simulink model "KUKA_main_simmechanic"  (R2015a)
settings: Solver=ode45  StartTime=0.0  StopTime=61.2  RelTol=1e-3
undefined symbols (not defined in the file or in its folder): KUKA, part1, part2, part3, part4, RootGround, RootPart, sfun3d
libraries: mblibv1 x16
settings Model: Creator=PHANTU  LastModifiedBy=PHANTU
settings SimMechanicsCC: VisOnUpdateDiagram=on  VisDuringSimulation=on

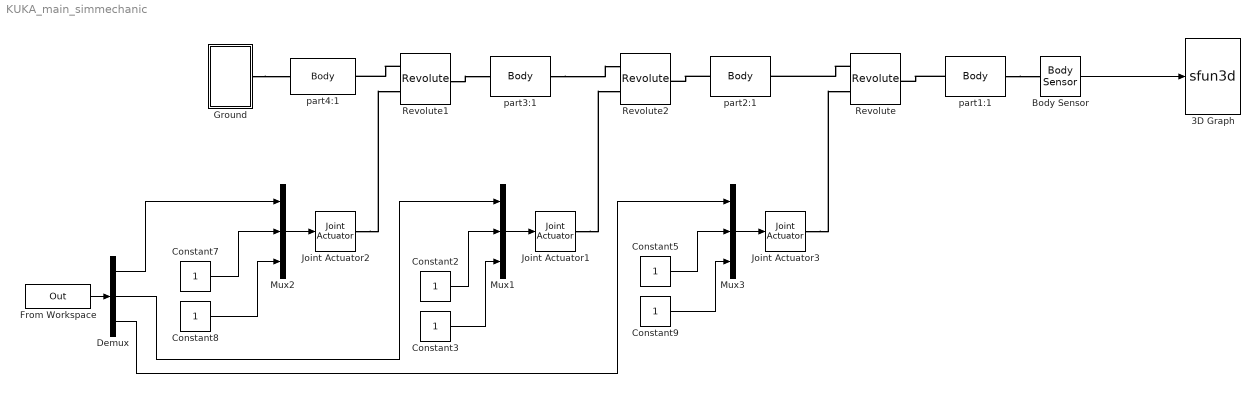
== system KUKA_main_simmechanic ==
  3D Graph : S-Function  LoadFcn=sfun3d([],[],[],'LoadBlock')  StartFcn=sfun3d([],[],[],'Start')  StopFcn=sfun3d([],[],[],'Stop')  FunctionName=sfun3d  Parameters=ax,T,np,cp,gd,ls,mk  mask(3D Graph){np=1, ax=[-50 800 -50 800 -100 800], cp=[40000 0 -50], gd=on, ls=-, mk=none, T=-1}
      mask prompts: np "Number of point (lines)"; ax "[xmin xmax  ymin ymax zmin zmax]"; cp "Camera position (use [0 0 1] for 2D XY view)"; gd "Grid (on|off)"; ls "LineStyle"; mk "Marker"; T "Sampling Time"
      mask help:
      | This block plots the position of several points in the XYZ space. The input contains the coordinates of all the points (x1,y1,z1,x2,y2,z2,...).
      | The number of points (lines), the XYZ ranges, camera position, grid, linestyle, marker and sampling time, can be set as mask parameters.
      settings: CopyFcn=sfun3d([],[],[],'CopyBlock')  DeleteFcn=sfun3d([],[],[],'DeleteBlock')  NameChangeFcn=sfun3d([],[],[],'NameChange')
      mask Help:
      | This block plots the position of several points in the XYZ space. The input contains the coordinates of all the points (x1,y1,z1,x2,y2,z2,...).
      | The number of points (lines), the XYZ ranges, camera position, grid, linestyle, marker and sampling time, can be set as mask parameters.
      mask TypeOptions ls: - | -- | : | -. | none
      mask TypeOptions mk: none | . | + | o | * | x | square | diamond | v | ^ | > | < | pentagram | hexagram
      mask Display: plot([.05 .95 .95 .05 .05],[.45 .45 .95 .95 .45], 0.5+cos(0:0.1:2*pi)*0.3,0.7+sin(0:0.1:2*pi)*0.2)
  Body Sensor : mblibv1/Sensors &  Actuators/Body Sensor  UpdateFromCAD=off  PhysicalDomain=Mechanical  PortType=blob  Muxed=on  Pose=off  Angle=on  AngleUnits=deg  ArcVelocity=off  ArcVelocityUnits=deg/s  ArcAcceleration=off  ArcAccelerationUnits=deg/s^2  CoordPosition=on  CoordPositionUnits=mm  Velocity=off  VelocityUnits=m/s  Acceleration=off  AccelerationUnits=m/s^2  Quaternion=on  QuaternionDT=off  QuaternionDDT=off  QuaternionUnits=off  OutputVector=[1]  ActiveIO=on  Width=3  DialogClass=MechanicalSensorBlock  ReferenceFrame=Absolute (World)
  Constant{2..3,5,7..9} (6 alike) : Constant
  Demux : Demux  Outputs=3
  From Workspace : FromWorkspace  VariableName=Out  SampleTime=0.1
  Ground : Subsystem
  Joint Actuator1 : mblibv1/Sensors &  Actuators/Joint Actuator  UpdateFromCAD=off  PhysicalDomain=Mechanical  PortType=blob  ActuationStyle=Motion  AngleUnits=deg  ArcVelocityUnits=deg/s  ArcAccelerationUnits=deg/s^2  CoordPositionUnits=m  VelocityUnits=m/s  AccelerationUnits=m/s^2  ForceUnits=N  TorqueUnits=N*m  ActiveIO=on  Width=3  DialogClass=MechanicalActuatorBlock  Primitive=R1  ReferenceFrame=Absolute (World)
  Joint Actuator2 : mblibv1/Sensors &  Actuators/Joint Actuator  UpdateFromCAD=off  PhysicalDomain=Mechanical  PortType=blob  ActuationStyle=Motion  AngleUnits=deg  ArcVelocityUnits=deg/s  ArcAccelerationUnits=deg/s^2  CoordPositionUnits=m  VelocityUnits=m/s  AccelerationUnits=m/s^2  ForceUnits=N  TorqueUnits=N*m  ActiveIO=on  Width=3  DialogClass=MechanicalActuatorBlock  Primitive=R1  ReferenceFrame=Absolute (World)
  Joint Actuator3 : mblibv1/Sensors &  Actuators/Joint Actuator  UpdateFromCAD=off  PhysicalDomain=Mechanical  PortType=blob  ActuationStyle=Motion  AngleUnits=deg  ArcVelocityUnits=deg/s  ArcAccelerationUnits=deg/s^2  CoordPositionUnits=m  VelocityUnits=m/s  AccelerationUnits=m/s^2  ForceUnits=N  TorqueUnits=N*m  ActiveIO=on  Width=3  DialogClass=MechanicalActuatorBlock  Primitive=R1  ReferenceFrame=Absolute (World)
  Mux1 : Mux  Inputs=3
  Mux2 : Mux  Inputs=3
  Mux3 : Mux  Inputs=3
  Revolute : mblibv1/Joints/Revolute  LConnTagsString=__newl0|SA1  RConnTagsString=__newr0  UpdateFromCAD=on  PMImportedID=part1:1:-:part2:1  NumSAPorts=1  CutJoint=off  MarkAsCut=off  Primitives=prismatic  PrimitiveProps=R1$World$[0,1,0]$revolute  DialogClass=JointBlock  R1Axis=[0,1,0]
  Revolute1 : mblibv1/Joints/Revolute  LConnTagsString=__newl0|SA1  RConnTagsString=__newr0  UpdateFromCAD=on  PMImportedID=part3:1:-:part4:1  NumSAPorts=1  CutJoint=off  MarkAsCut=off  Primitives=prismatic  PrimitiveProps=R1$World$[0,0,1]$revolute  DialogClass=JointBlock  R1Axis=[0,0,1]
  Revolute2 : mblibv1/Joints/Revolute  LConnTagsString=__newl0|SA1  RConnTagsString=__newr0  UpdateFromCAD=on  PMImportedID=part2:1:-:part3:1  NumSAPorts=1  CutJoint=off  MarkAsCut=off  Primitives=prismatic  PrimitiveProps=R1$World$[0,1,0]$revolute  DialogClass=JointBlock  R1Axis=[0,1,0]
  part1:1 : mblibv1/Bodies/Body  LConnTagsString=CS2  RConnTagsString=CS3  UpdateFromCAD=on  PMImportedID=part1:1  DialogClass=MechanicalBodyBlock  Mass=40.4989  MassUnits=kg  InertiaUnits=kg*m^2  Inertia=[0.772378,0.243082,0.407747;0.243082,3.65301,-0.170622;0.407747,-0.170622,3.50439]  Shape=Cylinder  ShapeDims=[1 1]  ShapeUnits=m  ShapeUse=false  Density=1  DensityUnits=kg/m^3  DensityUse=false  GraphicsMode=GFXFILE  GraphicsFileName=part1_ipt_86567821.STL  BodyColorSelMode=COLORPALETTE  BodyColor=[1;1;0]  AttachedToCS=CS1  CG=Right$CG$[1017.65 45.7629 740.059]$WORLD$WORLD$mm$[1 0 0;0 1 0;0 0 1]$3x3 Transform$rad$WORLD$false$part1:1::CG(AUTOGEN)  WorkingFrames=Right$CS1$[680 0 -679.99]$WORLD$WORLD$mm$[1 0 0;0 1 0;0 0 1]$3x3 Transform$rad$WORLD$false$part1:1::CS1(AUTOGEN)#Left$CS2$[940 -107 675.01]$WORLD$WORLD$mm$[1 0 0;0 1 0;0 0 1]$3x3 Transform$rad$WORLD$true$part1:1:-:part2:1::part1:1(AUTOGEN)#Right$CS3$[1768 0 675.01]$WORLD$WORLD$mm$[1 0 0;0 1 0;0 0 1]$3x3 Transform$rad$WORLD$true$none  CGPos=[1017.65 45.7629 740.059]  CGRot=[1 0 0;0 1 0;0 0 1]  CS0Pos=[]  CS0Rot=[]  CS1Pos=[680 0 -679.99]  CS1Rot=[1 0 0;0 1 0;0 0 1]  CS2Pos=[940 -107 675.01]  CS2Rot=[1 0 0;0 1 0;0 0 1]  CS3Pos=[1768 0 675.01]  CS3Rot=[1 0 0;0 1 0;0 0 1]  CS4Pos=[]  CS4Rot=[]  CS5Pos=[]  CS5Rot=[]  CS6Pos=[]  CS6Rot=[]  CS7Pos=[]  CS7Rot=[]  CS8Pos=[]  CS8Rot=[]  CS9Pos=[]  CS9Rot=[]  CS10Pos=[]  CS10Rot=[]  CS11Pos=[]  CS11Rot=[]  CS12Pos=[]  CS12Rot=[]  CS13Pos=[]  CS13Rot=[]  CS14Pos=[]  CS14Rot=[]  CS15Pos=[]  CS15Rot=[]  CS16Pos=[]  CS16Rot=[]  CS17Pos=[]  CS17Rot=[]  CS18Pos=[]  CS18Rot=[]  CS19Pos=[]  CS19Rot=[]  CS20Pos=[]  CS20Rot=[]
  part2:1 : mblibv1/Bodies/Body  LConnTagsString=CS3  RConnTagsString=CS2  UpdateFromCAD=on  PMImportedID=part2:1  DialogClass=MechanicalBodyBlock  Mass=13.5189  MassUnits=kg  InertiaUnits=kg*m^2  Inertia=[0.595755,-0.000241052,-0.000341583;-0.000241052,0.593927,0.0264066;-0.000341583,0.0264066,0.0592214]  Shape=Cylinder  ShapeDims=[1 1]  ShapeUnits=m  ShapeUse=false  Density=1  DensityUnits=kg/m^3  DensityUse=false  GraphicsMode=GFXFILE  GraphicsFileName=part2_ipt_86567821.STL  BodyColorSelMode=COLORPALETTE  BodyColor=[0;0;1]  AttachedToCS=CS1  CG=Right$CG$[581.389 -180.551 674.773]$WORLD$WORLD$mm$[0 0 1;0 1 0;-1 0 0]$3x3 Transform$rad$WORLD$false$part2:1::CG(AUTOGEN)  WorkingFrames=Right$CS1$[-415 0 935.01]$WORLD$WORLD$mm$[0 0 1;0 1 0;-1 0 0]$3x3 Transform$rad$WORLD$false$part2:1::CS1(AUTOGEN)#Right$CS2$[940 -107 675.01]$WORLD$WORLD$mm$[1 0 0;0 1 0;0 0 1]$3x3 Transform$rad$WORLD$true$part1:1:-:part2:1::part2:1(AUTOGEN)#Left$CS3$[260 -83 675.01]$WORLD$WORLD$mm$[1 0 0;0 1 0;0 0 1]$3x3 Transform$rad$WORLD$true$part2:1:-:part3:1::part2:1(AUTOGEN)  CGPos=[581.389 -180.551 674.773]  CGRot=[0 0 1;0 1 0;-1 0 0]  CS0Pos=[]  CS0Rot=[]  CS1Pos=[-415 0 935.01]  CS1Rot=[0 0 1;0 1 0;-1 0 0]  CS2Pos=[940 -107 675.01]  CS2Rot=[1 0 0;0 1 0;0 0 1]  CS3Pos=[260 -83 675.01]  CS3Rot=[1 0 0;0 1 0;0 0 1]  CS4Pos=[]  CS4Rot=[]  CS5Pos=[]  CS5Rot=[]  CS6Pos=[]  CS6Rot=[]  CS7Pos=[]  CS7Rot=[]  CS8Pos=[]  CS8Rot=[]  CS9Pos=[]  CS9Rot=[]  CS10Pos=[]  CS10Rot=[]  CS11Pos=[]  CS11Rot=[]  CS12Pos=[]  CS12Rot=[]  CS13Pos=[]  CS13Rot=[]  CS14Pos=[]  CS14Rot=[]  CS15Pos=[]  CS15Rot=[]  CS16Pos=[]  CS16Rot=[]  CS17Pos=[]  CS17Rot=[]  CS18Pos=[]  CS18Rot=[]  CS19Pos=[]  CS19Rot=[]  CS20Pos=[]  CS20Rot=[]
  part3:1 : mblibv1/Bodies/Body  LConnTagsString=CS2  RConnTagsString=CS3  UpdateFromCAD=on  PMImportedID=part3:1  DialogClass=MechanicalBodyBlock  Mass=28.3532  MassUnits=kg  InertiaUnits=kg*m^2  Inertia=[1.07185,-0.0539717,-0.354129;-0.0539717,1.05703,-0.0608066;-0.354129,-0.0608066,1.30191]  Shape=Cylinder  ShapeDims=[1 1]  ShapeUnits=m  ShapeUse=false  Density=1  DensityUnits=kg/m^3  DensityUse=false  GraphicsMode=GFXFILE  GraphicsFileName=part3_ipt_86567821.STL  BodyColorSelMode=COLORPALETTE  BodyColor=[1;0.843137;0]  AttachedToCS=CS1  CG=Right$CG$[107.444 17.0185 548.784]$WORLD$WORLD$mm$[1 0 0;0 1 0;0 0 1]$3x3 Transform$rad$WORLD$false$part3:1::CG(AUTOGEN)  WorkingFrames=Right$CS1$[0 0 0.00950136]$WORLD$WORLD$mm$[1 0 0;0 1 0;0 0 1]$3x3 Transform$rad$WORLD$false$part3:1::CS1(AUTOGEN)#Left$CS2$[0 0 396.933]$WORLD$WORLD$mm$[1 0 0;0 1 0;0 0 1]$3x3 Transform$rad$WORLD$true$part3:1:-:part4:1::part3:1(AUTOGEN)#Right$CS3$[260 -83 675.01]$WORLD$WORLD$mm$[1 0 0;0 1 0;0 0 1]$3x3 Transform$rad$WORLD$true$part2:1:-:part3:1::part3:1(AUTOGEN)  CGPos=[107.444 17.0185 548.784]  CGRot=[1 0 0;0 1 0;0 0 1]  CS0Pos=[]  CS0Rot=[]  CS1Pos=[0 0 0.00950136]  CS1Rot=[1 0 0;0 1 0;0 0 1]  CS2Pos=[0 0 396.933]  CS2Rot=[1 0 0;0 1 0;0 0 1]  CS3Pos=[260 -83 675.01]  CS3Rot=[1 0 0;0 1 0;0 0 1]  CS4Pos=[]  CS4Rot=[]  CS5Pos=[]  CS5Rot=[]  CS6Pos=[]  CS6Rot=[]  CS7Pos=[]  CS7Rot=[]  CS8Pos=[]  CS8Rot=[]  CS9Pos=[]  CS9Rot=[]  CS10Pos=[]  CS10Rot=[]  CS11Pos=[]  CS11Rot=[]  CS12Pos=[]  CS12Rot=[]  CS13Pos=[]  CS13Rot=[]  CS14Pos=[]  CS14Rot=[]  CS15Pos=[]  CS15Rot=[]  CS16Pos=[]  CS16Rot=[]  CS17Pos=[]  CS17Rot=[]  CS18Pos=[]  CS18Rot=[]  CS19Pos=[]  CS19Rot=[]  CS20Pos=[]  CS20Rot=[]
  part4:1 : mblibv1/Bodies/Body  LConnTagsString=CS2  RConnTagsString=CS3  UpdateFromCAD=on  PMImportedID=part4:1  DialogClass=MechanicalBodyBlock  Mass=69.1518  MassUnits=kg  InertiaUnits=kg*m^2  Inertia=[1.73395,-0.0485512,-0.0688783;-0.0485512,2.09396,-0.000359291;-0.0688783,-0.000359291,2.19578]  Shape=Cylinder  ShapeDims=[1 1]  ShapeUnits=m  ShapeUse=false  Density=1  DensityUnits=kg/m^3  DensityUse=false  GraphicsMode=GFXFILE  GraphicsFileName=part4_ipt_86567821.STL  BodyColorSelMode=COLORPALETTE  BodyColor=[1;0;0]  AttachedToCS=CS1  CG=Right$CG$[-41.1494 -3.79313 198.366]$WORLD$WORLD$mm$[1 0 0;0 1 0;0 0 1]$3x3 Transform$rad$WORLD$false$part4:1::CG(AUTOGEN)  WorkingFrames=Right$CS1$[0.557964 0.1152 -1.667]$WORLD$WORLD$mm$[1 0 0;0 1 0;0 0 1]$3x3 Transform$rad$WORLD$false$part4:1::CS1(AUTOGEN)#Left$CS2$[0 0 0]$WORLD$WORLD$mm$[1 0 0;0 1 0;0 0 1]$3x3 Transform$rad$WORLD$true$:-:KUKA/RootPart::part4:1(AUTOGEN)#Right$CS3$[0 0 396.933]$WORLD$WORLD$mm$[1 0 0;0 1 0;0 0 1]$3x3 Transform$rad$WORLD$true$part3:1:-:part4:1::part4:1(AUTOGEN)  CGPos=[-41.1494 -3.79313 198.366]  CGRot=[1 0 0;0 1 0;0 0 1]  CS0Pos=[]  CS0Rot=[]  CS1Pos=[0.557964 0.1152 -1.667]  CS1Rot=[1 0 0;0 1 0;0 0 1]  CS2Pos=[0 0 0]  CS2Rot=[1 0 0;0 1 0;0 0 1]  CS3Pos=[0 0 396.933]  CS3Rot=[1 0 0;0 1 0;0 0 1]  CS4Pos=[]  CS4Rot=[]  CS5Pos=[]  CS5Rot=[]  CS6Pos=[]  CS6Rot=[]  CS7Pos=[]  CS7Rot=[]  CS8Pos=[]  CS8Rot=[]  CS9Pos=[]  CS9Rot=[]  CS10Pos=[]  CS10Rot=[]  CS11Pos=[]  CS11Rot=[]  CS12Pos=[]  CS12Rot=[]  CS13Pos=[]  CS13Rot=[]  CS14Pos=[]  CS14Rot=[]  CS15Pos=[]  CS15Rot=[]  CS16Pos=[]  CS16Rot=[]  CS17Pos=[]  CS17Rot=[]  CS18Pos=[]  CS18Rot=[]  CS19Pos=[]  CS19Rot=[]  CS20Pos=[]  CS20Rot=[]
  wires:
  Mux2/1 -> Joint Actuator2/1
  Constant7/1 -> Mux2/2
  Constant8/1 -> Mux2/3
  Mux1/1 -> Joint Actuator1/1
  Constant2/1 -> Mux1/2
  Constant3/1 -> Mux1/3
  Mux3/1 -> Joint Actuator3/1
  Constant5/1 -> Mux3/2
  Constant9/1 -> Mux3/3
  From Workspace/1 -> Demux/1
  Demux/1 -> Mux2/1
  Demux/2 -> Mux1/1
  Demux/3 -> Mux3/1
  Body Sensor/1 -> 3D Graph/1
  connections:
  Revolute1/LConn1 -- part4:1/RConn1
  Revolute1/RConn1 -- part3:1/LConn1
  part3:1/RConn1 -- Revolute2/LConn1
  Revolute/LConn1 -- part2:1/RConn1
  part2:1/LConn1 -- Revolute2/RConn1
  part1:1/LConn1 -- Revolute/RConn1
  Ground/RConn1 -- part4:1/LConn1
  Joint Actuator2/RConn1 -- Revolute1/LConn2
  Joint Actuator1/RConn1 -- Revolute2/LConn2
  Joint Actuator3/RConn1 -- Revolute/LConn2
  part1:1/RConn1 -- Body Sensor/LConn1

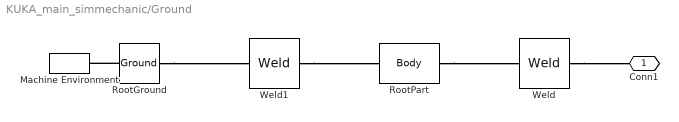
== system KUKA_main_simmechanic/Ground ==
  Machine Environment : mblibv1/Bodies/Machine Environment  PortType=env  PhysicalDomain=Mechanical  DialogTemplateClass=MECH.MachineEnvironment  SyncWhenCopied=off  Gravity=[0 0 -9.81]  GravityUnits=m/s^2  GravityAsSignal=off  Dimensionality=Auto-detect  AnalysisType=Forward dynamics  LinearAssemblyTolerance=1e-3  LinearAssemblyToleranceUnits=m  AngularAssemblyTolerance=1e-3  AngularAssemblyToleranceUnits=rad  ConstraintSolverType=Stabilizing  ConstraintRelTolerance=1e-4  ConstraintAbsTolerance=1e-4  UseRobustSingularityHandling=off  RedundancyAnalysisToleranceType=Automatically select tolerance  RedundancyAnalysisTolerance=1e-14  StatePerturbationType=Fixed  PerturbationSize=1e-5  VisualizeMachine=on  BodyVisualizationType=Use model default body geometries  BodyColorSelMode=Use model default  DefaultBodyColor=[1 0 0]
  RootGround : mblibv1/Bodies/Ground  UpdateFromCAD=on  PMImportedID=RootGround  LeftPortType=env  RightPortType=workingframe  PhysicalDomain=Mechanical  DialogClass=GroundBlock  CoordPosition=[325.194,-2.42393,451.225]  CoordPositionUnits=mm  StateVectorMgrId=0  MachineId=[1 0]  ShowEnvPort=on  ParameterChecksum=[4075420938, 176014192, 2168610692, 345075913]  TopologyChecksum=[3153187368, 2124946678, 2062417528, 4113742079]
  RootPart : mblibv1/Bodies/Body  LConnTagsString=CS3  RConnTagsString=CS2  UpdateFromCAD=on  PMImportedID=KUKA/RootPart  DialogClass=MechanicalBodyBlock  Mass=0  MassUnits=kg  InertiaUnits=kg*m^2  Inertia=[0,0,0;0,0,0;0,0,0]  Shape=Cylinder  ShapeDims=[1 1]  ShapeUnits=m  ShapeUse=false  Density=1  DensityUnits=kg/m^3  DensityUse=false  GraphicsMode=MACHINE_DEFAULT  BodyColorSelMode=MACHINE_DEFAULT  BodyColor=[1;0;0]  AttachedToCS=CS1  CG=Right$CG$[325.194 -2.42393 451.225]$WORLD$WORLD$mm$[1 0 0;0 1 0;0 0 1]$3x3 Transform$rad$WORLD$false$KUKA/RootPart::CG(AUTOGEN)  WorkingFrames=Right$CS1$[0 0 0]$WORLD$WORLD$mm$[1 0 0;0 1 0;0 0 1]$3x3 Transform$rad$WORLD$false$KUKA/RootPart::CS1(AUTOGEN)#Right$CS2$[0 0 0]$WORLD$WORLD$mm$[1 0 0;0 1 0;0 0 1]$3x3 Transform$rad$WORLD$true$:-:KUKA/RootPart::KUKA/RootPart(AUTOGEN)#Left$CS3$[325.194 -2.42393 451.225]$WORLD$WORLD$mm$[1 0 0;0 1 0;0 0 1]$3x3 Transform$rad$WORLD$true$KUKA/RootPart:-:RootGround::KUKA/RootPart(AUTOGEN)  CGPos=[325.194 -2.42393 451.225]  CGRot=[1 0 0;0 1 0;0 0 1]  CS0Pos=[]  CS0Rot=[]  CS1Pos=[0 0 0]  CS1Rot=[1 0 0;0 1 0;0 0 1]  CS2Pos=[0 0 0]  CS2Rot=[1 0 0;0 1 0;0 0 1]  CS3Pos=[325.194 -2.42393 451.225]  CS3Rot=[1 0 0;0 1 0;0 0 1]  CS4Pos=[]  CS4Rot=[]  CS5Pos=[]  CS5Rot=[]  CS6Pos=[]  CS6Rot=[]  CS7Pos=[]  CS7Rot=[]  CS8Pos=[]  CS8Rot=[]  CS9Pos=[]  CS9Rot=[]  CS10Pos=[]  CS10Rot=[]  CS11Pos=[]  CS11Rot=[]  CS12Pos=[]  CS12Rot=[]  CS13Pos=[]  CS13Rot=[]  CS14Pos=[]  CS14Rot=[]  CS15Pos=[]  CS15Rot=[]  CS16Pos=[]  CS16Rot=[]  CS17Pos=[]  CS17Rot=[]  CS18Pos=[]  CS18Rot=[]  CS19Pos=[]  CS19Rot=[]  CS20Pos=[]  CS20Rot=[]
  Weld : mblibv1/Joints/Weld  LConnTagsString=__newl0  RConnTagsString=__newr0  UpdateFromCAD=on  PMImportedID=:-:KUKA/RootPart  NumSAPorts=0  CutJoint=off  MarkAsCut=off  Primitives=weld  PrimitiveProps=W$WORLD$[0.57735,0.57735,0.57735]$weld  DialogClass=JointBlock  WAxis=[0.57735,0.57735,0.57735]
  Weld1 : mblibv1/Joints/Weld  LConnTagsString=__newl0  RConnTagsString=__newr0  UpdateFromCAD=on  PMImportedID=KUKA/RootPart:-:RootGround  NumSAPorts=0  CutJoint=off  MarkAsCut=off  Primitives=weld  PrimitiveProps=W$WORLD$[0.57735,0.57735,0.57735]$weld  DialogClass=JointBlock  WAxis=[0.57735,0.57735,0.57735]
  Conn1 : PMIOPort  Port=1  Side=Right
  connections:
  Weld/RConn1 -- Conn1/RConn1
  RootPart/RConn1 -- Weld/LConn1
  RootGround/RConn1 -- Weld1/LConn1
  Weld1/RConn1 -- RootPart/LConn1
  RootGround/LConn1 -- Machine Environment/RConn1
